simulink model "BatteryManagementSystem_V1"  (R2024a)
settings: Solver=VariableStepAuto  StartTime=0.0  StopTime=3600*2  RelTol=1e-3
InitFcn:
  | Capacity = 2.65;
  | c_rate= 0.5;
  | Np = 1; % Number of parallel cells
  | Ns = 3; % Number of series cells
  | voltageMin= 3.2;
  | currentThreshold = Capacity*Np/30;
  | voltageThreshold = 4.3;
  | CV_gain = 1;
  | voltageTolerance = 2;
undefined symbols (not defined in the file or in its folder): DiscIntNeverNeededParam
settings Model: Creator=MANSY  LastModifiedBy=MANSY
settings OptimizationCC: DefaultParameterBehavior=Inlined  UseDivisionForNetSlopeComputation=on  GainParamInheritBuiltInType=on  UseFloatMulNetSlope=on  InlineInvariantSignals=on  PassReuseOutputArgsAs=Individual arguments  ZeroExternalMemoryAtStartup=off  ZeroInternalMemoryAtStartup=off  NoFixptDivByZeroProtection=on  EfficientFloat2IntCast=on  LifeSpan=1  OptimizeBlockOrder=speed  DifferentSizesBufferReuse=on  EfficientTunableParamExpr=on
settings DebuggingCC: ParameterTunabilityLossMsg=error
settings HardwareCC: ProdBitPerInt=16  ProdBitPerPointer=16  ProdBitPerSizeT=16  ProdBitPerPtrDiffT=16  ProdLargestAtomicFloat=None  ProdWordSize=8  ProdLongLongMode=on  ProdHWDeviceType=Atmel->AVR
settings SFSimCC: MATLABDynamicMemAlloc=off
settings RTWCC: Description=Embedded Coder  SystemTargetFile=ert.tlc  TemplateMakefile=ert_default_tmf  PortableWordSizes=on
settings CodeAppCC: ForceParamTrailComments=on  IgnoreCustomStorageClasses=off  OperatorAnnotations=on  SimulinkDataObjDesc=on  SFDataObjDesc=on  CustomSymbolStrGlobalVar=rt$N$M  CustomSymbolStrType=$N$M  CustomSymbolStrFcn=$N$M$F  CustomSymbolStrMacro=$N$M  InsertBlockDesc=on
settings ERTTargetCC: TargetLangStandard=C99 (ISO)  GenerateSampleERTMain=on  IncludeMdlTerminateFcn=off  CombineSignalStateStructs=on  SupportComplex=off  SupportNonInlinedSFcns=on  InlinedParameterPlacement=NonHierarchical  ERTCustomFileTemplate=example_file_process.tlc  ERTFilePackagingFormat=CompactWithDataFile

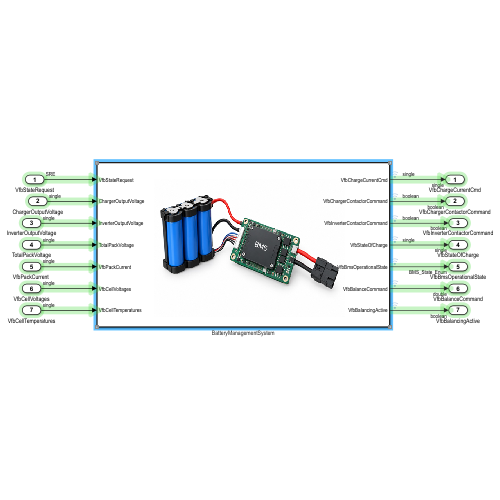
[thumbnail: Simulink's stored preview of the top-level diagram]
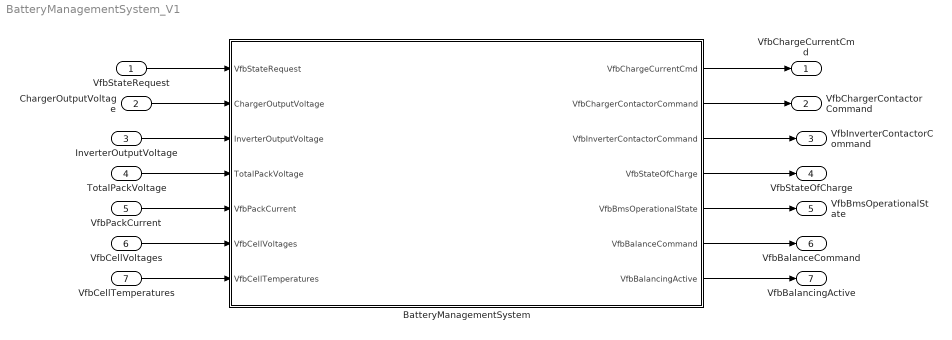
== system BatteryManagementSystem_V1 ==
  VfbStateRequest : Inport
  ChargerOutputVoltage : Inport  Port=2
  InverterOutputVoltage : Inport  Port=3
  TotalPackVoltage : Inport  Port=4
  "VfbPackCurrent " : Inport  Port=5
  VfbCellVoltages : Inport  Port=6
  VfbCellTemperatures : Inport  Port=7
  BatteryManagementSystem : Subsystem  TreatAsAtomicUnit=on
      mask Display: image('Lithium-Ion Battery BMS Module.png');
  VfbChargeCurrentCmd : Outport  OutDataTypeStr=single
  VfbChargerContactorCommand : Outport  Port=2  OutDataTypeStr=boolean
  VfbInverterContactorCommand : Outport  Port=3  OutDataTypeStr=boolean
  VfbStateOfCharge : Outport  Port=4  OutDataTypeStr=single
  VfbBmsOperationalState : Outport  Port=5
  VfbBalanceCommand : Outport  Port=6
  VfbBalancingActive : Outport  Port=7
  wires:
  VfbStateRequest/1 -> BatteryManagementSystem/1(VfbStateRequest)
  ChargerOutputVoltage/1 -> BatteryManagementSystem/2(ChargerOutputVoltage)
  InverterOutputVoltage/1 -> BatteryManagementSystem/3(InverterOutputVoltage)
  TotalPackVoltage/1 -> BatteryManagementSystem/4(TotalPackVoltage)
  "VfbPackCurrent "/1 -> BatteryManagementSystem/5("VfbPackCurrent ")
  VfbCellVoltages/1 -> BatteryManagementSystem/6(VfbCellVoltages)
  VfbCellTemperatures/1 -> BatteryManagementSystem/7(VfbCellTemperatures)
  BatteryManagementSystem/1(VfbChargeCurrentCmd) -> VfbChargeCurrentCmd/1
  BatteryManagementSystem/2(VfbChargerContactorCommand) -> VfbChargerContactorCommand/1
  BatteryManagementSystem/3(VfbInverterContactorCommand) -> VfbInverterContactorCommand/1
  BatteryManagementSystem/5(VfbBmsOperationalState) -> VfbBmsOperationalState/1
  BatteryManagementSystem/4(VfbStateOfCharge) -> VfbStateOfCharge/1
  BatteryManagementSystem/6(VfbBalanceCommand) -> VfbBalanceCommand/1
  BatteryManagementSystem/7(VfbBalancingActive) -> VfbBalancingActive/1

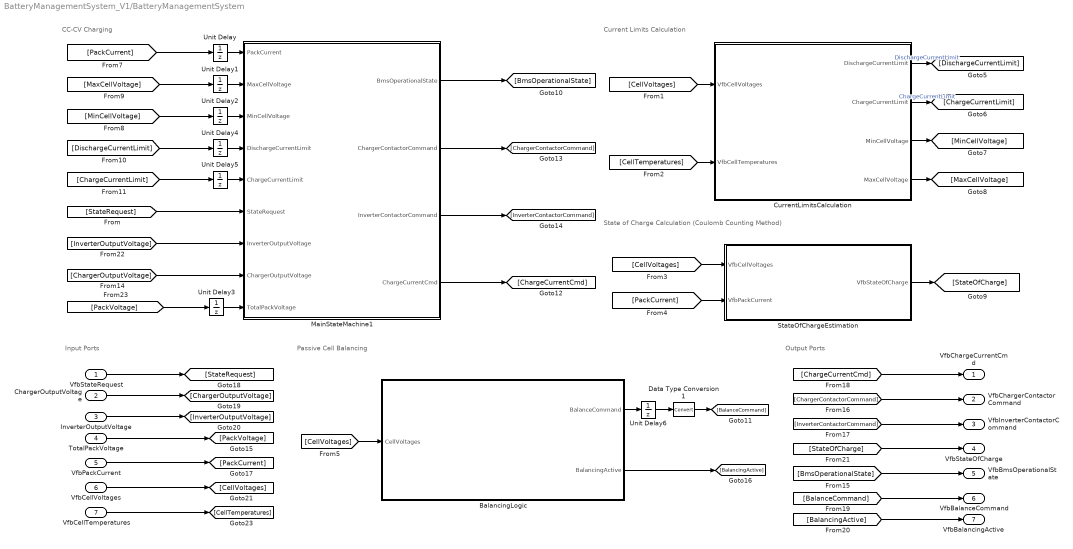
== system BatteryManagementSystem_V1/BatteryManagementSystem ==
  note: Passive Cell Balancing
  note: State of Charge Calculation (Coulomb Counting Method)
  note: Current Limits Calculation
  note: CC-CV Charging
  note: Output Ports
  note: Input Ports
  VfbStateRequest : Inport
  ChargerOutputVoltage : Inport  Port=2
  InverterOutputVoltage : Inport  Port=3
  TotalPackVoltage : Inport  Port=4
  "VfbPackCurrent " : Inport  Port=5
  VfbCellVoltages : Inport  Port=6
  VfbCellTemperatures : Inport  Port=7
  " StateOfChargeEstimation" : Subsystem  TreatAsAtomicUnit=on  SystemSampleTime=200e-3
      mask Display: image('SOC_img.png');
  BalancingLogic : MATLAB Function  TreatAsAtomicUnit=on  SystemSampleTime=250e-3
  "CurrentLimitsCalculation " : Subsystem  TreatAsAtomicUnit=on  SystemSampleTime=100e-3
      mask Display: image('CurrentLimit_img.png');
  Data Type Conversion1 : DataTypeConversion  SaturateOnIntegerOverflow=off  RndMeth=Floor
  MainStateMachine1 : Stateflow chart  TreatAsAtomicUnit=on  SystemSampleTime=50e-3
      settings: PortSchema="{\"entries\":[{\"content\":{\"sides\":[{\"content\":{\"connectorIds\":[\"In1\",\"In2\",\"In3\",\"In5\",\"In4\",\"In6\",\"In8\",\"In7\",\"In9\"]},\"type\":\"ConnectorPlacement.EquallySpacedRectSide\",\"uuid\":\"093f55e8-f90e-4d40-b8fb-904662301821\"},{\"content\":{\"connectorIds\":[\"Out1\",\"Out2\",\"Out3\",\"Out4\"],\"side\":\"RIGHT\"},\"type\":\"ConnectorPlacement.EquallySpacedRectSide\",\"uuid\":\"5101bd8f-b6b7-43f5-a647-8a1816a9003d\"},{\"content\":{\"side\":\"TOP\"},\"type\":\"ConnectorPlacement.EquallySpacedRectSide\",\"uuid\":\"c14aa96a-7f57-47da-866c-602a285b1131\"}]},\"type\":\"ConnectorPlacement.EquallySpacedConnector\",\"uuid\":\"8109f1a5-bcb4-40d5-94fc-489b7534b704\"}],\"packageUris\":[\"http://schema.mathworks.com/mf0/Connector/R2020b\"],\"version\":\"1.0\"}"
  Unit Delay{,1..6} (7 alike) : UnitDelay  SampleTime=-1  HasFrameUpgradeWarning=on
  VfbChargeCurrentCmd : Outport  OutDataTypeStr=single
  VfbChargerContactorCommand : Outport  Port=2  OutDataTypeStr=boolean
  VfbInverterContactorCommand : Outport  Port=3  OutDataTypeStr=boolean
  VfbStateOfCharge : Outport  Port=4  OutDataTypeStr=single
  VfbBmsOperationalState : Outport  Port=5
  VfbBalanceCommand : Outport  Port=6
  VfbBalancingActive : Outport  Port=7
  wires:
  TotalPackVoltage/1 -> [PackVoltage]
  MainStateMachine1/3(InverterContactorCommand) -> [InverterContactorCommand]
  [CellVoltages] -> "CurrentLimitsCalculation "/1(VfbCellVoltages)
  [BalancingActive] -> VfbBalancingActive/1
  "VfbPackCurrent "/1 -> [PackCurrent]
  "CurrentLimitsCalculation "/4(MaxCellVoltage) -> [MaxCellVoltage]
  [StateOfCharge] -> VfbStateOfCharge/1
  [InverterContactorCommand] -> VfbInverterContactorCommand/1
  [PackCurrent] -> Unit Delay/1
  MainStateMachine1/4(ChargeCurrentCmd) -> [ChargeCurrentCmd]
  Unit Delay5/1 -> MainStateMachine1/4(ChargeCurrentLimit)
  Data Type Conversion1/1 -> [BalanceCommand]
  [BalanceCommand] -> VfbBalanceCommand/1
  [ChargerContactorCommand] -> VfbChargerContactorCommand/1
  [InverterOutputVoltage] -> MainStateMachine1/8(InverterOutputVoltage)
  Unit Delay3/1 -> MainStateMachine1/9(TotalPackVoltage)
  [BmsOperationalState] -> VfbBmsOperationalState/1
  [StateRequest] -> MainStateMachine1/6(StateRequest)
  BalancingLogic/1(BalanceCommand) -> Unit Delay6/1
  BalancingLogic/2(BalancingActive) -> [BalancingActive]
  [DischargeCurrentLimit] -> Unit Delay4/1
  [ChargeCurrentCmd] -> VfbChargeCurrentCmd/1
  [ChargerOutputVoltage] -> MainStateMachine1/7(ChargerOutputVoltage)
  [ChargeCurrentLimit] -> Unit Delay5/1
  Unit Delay/1 -> MainStateMachine1/1(PackCurrent)
  Unit Delay1/1 -> MainStateMachine1/2(MaxCellVoltage)
  [CellTemperatures] -> "CurrentLimitsCalculation "/2(VfbCellTemperatures)
  [PackCurrent] -> " StateOfChargeEstimation"/2("VfbPackCurrent ")
  InverterOutputVoltage/1 -> [InverterOutputVoltage]
  Unit Delay6/1 -> Data Type Conversion1/1
  MainStateMachine1/2(ChargerContactorCommand) -> [ChargerContactorCommand]
  [MaxCellVoltage] -> Unit Delay1/1
  VfbCellVoltages/1 -> [CellVoltages]
  [PackVoltage] -> Unit Delay3/1
  VfbCellTemperatures/1 -> [CellTemperatures]
  [CellVoltages] -> BalancingLogic/1(CellVoltages)
  [CellVoltages] -> " StateOfChargeEstimation"/1(VfbCellVoltages)
  MainStateMachine1/1(BmsOperationalState) -> [BmsOperationalState]
  [MinCellVoltage] -> Unit Delay2/1
  "CurrentLimitsCalculation "/2(ChargeCurrentLimit) -> [ChargeCurrentLimit]  "ChargeCurrentLimit"
  ChargerOutputVoltage/1 -> [ChargerOutputVoltage]
  "CurrentLimitsCalculation "/1(DischargeCurrentLimit) -> [DischargeCurrentLimit]  "DischargeCurrentLimit"
  " StateOfChargeEstimation"/1(VfbStateOfCharge) -> [StateOfCharge]
  Unit Delay4/1 -> MainStateMachine1/5(DischargeCurrentLimit)
  VfbStateRequest/1 -> [StateRequest]
  Unit Delay2/1 -> MainStateMachine1/3(MinCellVoltage)
  "CurrentLimitsCalculation "/3(MinCellVoltage) -> [MinCellVoltage]

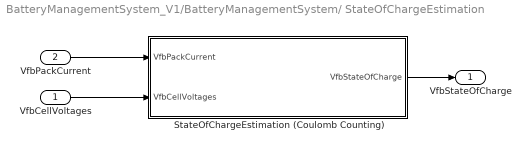
== system BatteryManagementSystem_V1/BatteryManagementSystem/ StateOfChargeEstimation ==
  VfbCellVoltages : Inport
  "VfbPackCurrent " : Inport  Port=2
  StateOfChargeEstimation (Coulomb Counting) : Subsystem  TreatAsAtomicUnit=on
  VfbStateOfCharge : Outport
  wires:
  StateOfChargeEstimation (Coulomb Counting)/1(VfbStateOfCharge) -> VfbStateOfCharge/1
  "VfbPackCurrent "/1 -> StateOfChargeEstimation (Coulomb Counting)/1("VfbPackCurrent ")
  VfbCellVoltages/1 -> StateOfChargeEstimation (Coulomb Counting)/2(VfbCellVoltages)

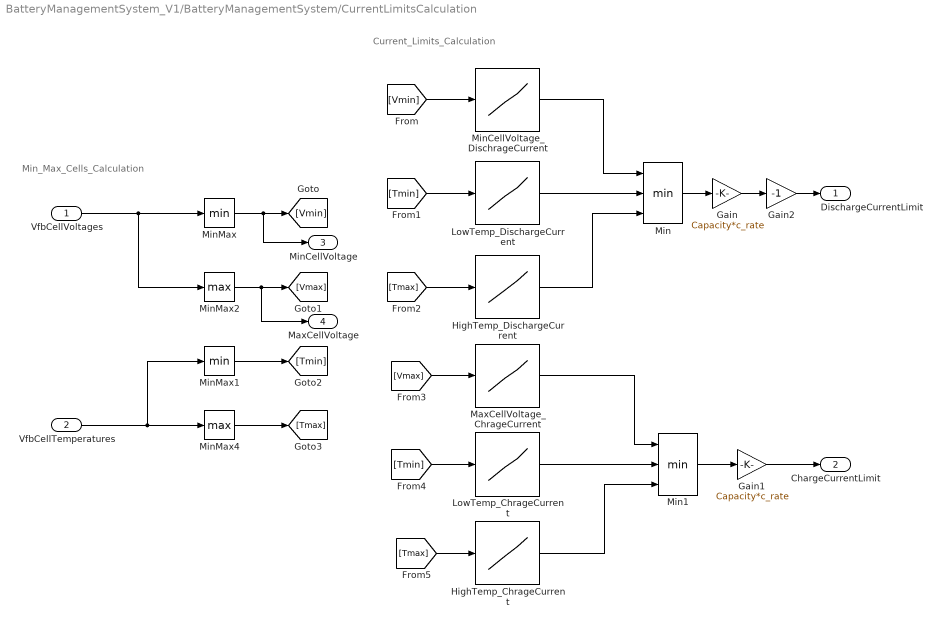
== system BatteryManagementSystem_V1/BatteryManagementSystem/CurrentLimitsCalculation  ==
  note: Current_Limits_Calculation
  note: Min_Max_Cells_Calculation
  VfbCellVoltages : Inport  OutDataTypeStr=single  PortDimensions=3
  VfbCellTemperatures : Inport  Port=2  OutDataTypeStr=single  PortDimensions=3
  Gain : Gain  Gain=Capacity*c_rate
  Gain1 : Gain  Gain=Capacity*c_rate
  Gain2 : Gain  Gain=-1
  HighTemp_ChrageCurrent : Lookup_n-D  NumberOfTableDimensions=1  BreakpointsForDimension1=single([298.15 308.15 313.15 318.15 323.15 333.15])  Table=single([1 1 0.8 0.5 0.2 0])  InternalRulePriority=Speed  RndMeth=Simplest
  HighTemp_DischargeCurrent : Lookup_n-D  NumberOfTableDimensions=1  BreakpointsForDimension1=single([298.15 308.15 313.15 318.15 323.15 333.15])  Table=single([1 1 0.9 0.7 0.4 0])  InternalRulePriority=Speed  RndMeth=Simplest
  LowTemp_ChrageCurrent : Lookup_n-D  NumberOfTableDimensions=1  BreakpointsForDimension1=single([243.15 263.15 273.15 278.15 283.15 288.15 298.15])  Table=single([0 0 0 0.1 0.3 0.6 1])  InternalRulePriority=Speed  RndMeth=Simplest
  LowTemp_DischargeCurrent : Lookup_n-D  NumberOfTableDimensions=1  BreakpointsForDimension1=single([243.15 258.15 273.15 283.15 293.15 298.15])  Table=single([0 0 0.2 0.6 0.9 1])  InternalRulePriority=Speed  RndMeth=Simplest
  MaxCellVoltage_ChrageCurrent : Lookup_n-D  NumberOfTableDimensions=1  BreakpointsForDimension1=single([3.0 3.5 3.8 4.0 4.1 4.2 4.25 4.35])  Table=single([1 1 1 0.9 0.7 0.4 0.2 0])  InternalRulePriority=Speed  RndMeth=Simplest
  Min : MinMax  Inputs=3
  Min1 : MinMax  Inputs=3
  MinCellVoltage_DischrageCurrent : Lookup_n-D  NumberOfTableDimensions=1  BreakpointsForDimension1=single([2.7 2.8 3.0 3.2 3.4 3.6])  Table=single([0 0.1 0.3 0.6 0.9 1])  InternalRulePriority=Speed  RndMeth=Simplest
  MinMax : MinMax
  MinMax1 : MinMax
  MinMax2 : MinMax  Function=max
  MinMax4 : MinMax  Function=max
  DischargeCurrentLimit : Outport  OutDataTypeStr=single
  ChargeCurrentLimit : Outport  Port=2  OutDataTypeStr=single
  MinCellVoltage : Outport  Port=3
  MaxCellVoltage : Outport  Port=4
  wires:
  [Vmin] -> MinCellVoltage_DischrageCurrent/1
  Gain/1 -> Gain2/1
  VfbCellVoltages/1 -> MinMax2/1, MinMax/1
  LowTemp_ChrageCurrent/1 -> Min1/2
  [Tmin] -> LowTemp_ChrageCurrent/1
  MinMax4/1 -> [Tmax]
  [Tmin] -> LowTemp_DischargeCurrent/1
  [Tmax] -> HighTemp_ChrageCurrent/1
  Min1/1 -> Gain1/1
  MaxCellVoltage_ChrageCurrent/1 -> Min1/1
  MinMax/1 -> MinCellVoltage/1, [Vmin]
  LowTemp_DischargeCurrent/1 -> Min/2
  MinMax2/1 -> MaxCellVoltage/1, [Vmax]
  HighTemp_DischargeCurrent/1 -> Min/3
  HighTemp_ChrageCurrent/1 -> Min1/3
  Gain1/1 -> ChargeCurrentLimit/1
  [Tmax] -> HighTemp_DischargeCurrent/1
  Min/1 -> Gain/1
  [Vmax] -> MaxCellVoltage_ChrageCurrent/1
  MinCellVoltage_DischrageCurrent/1 -> Min/1
  VfbCellTemperatures/1 -> MinMax4/1, MinMax1/1
  MinMax1/1 -> [Tmin]
  Gain2/1 -> DischargeCurrentLimit/1

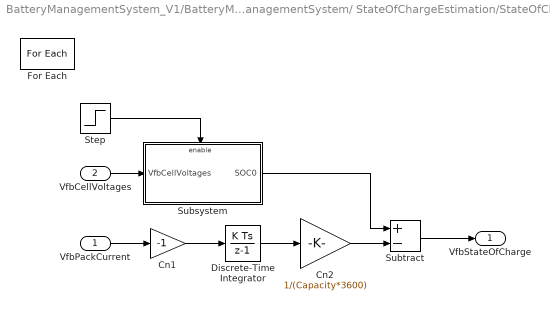
== system BatteryManagementSystem_V1/BatteryManagementSystem/ StateOfChargeEstimation/StateOfChargeEstimation (Coulomb Counting) ==
  "VfbPackCurrent " : Inport  OutDataTypeStr=single
  VfbCellVoltages : Inport  Port=2  Partition=on  PartitionDimension=1  PartitionWidth=1  PartitionOffset=0
  Cn1 : Gain  Gain=-1  OutDataTypeStr=single
  Cn2 : Gain  Gain=1/(Capacity*3600)  OutDataTypeStr=single
  Discrete-Time Integrator : DiscreteIntegrator  gainval=1  SampleTime=-1  OutDataTypeStr=single  RndMeth=Nearest  ICPrevOutput=DiscIntNeverNeededParam  ICPrevScaledInput=DiscIntNeverNeededParam
  For Each : ForEach  DisableCoverage=on
  Step : Step  Time=0.1  Before=1  After=0
  Subsystem : Subsystem
  Subtract : Sum  Inputs=+-
  VfbStateOfCharge : Outport  OutDataTypeStr=single  ConcatenationDimension=1
  wires:
  Cn1/1 -> Discrete-Time Integrator/1
  Discrete-Time Integrator/1 -> Cn2/1
  "VfbPackCurrent "/1 -> Cn1/1
  Subtract/1 -> VfbStateOfCharge/1
  Subsystem/1(SOC0) -> Subtract/1
  Step/1 -> Subsystem/Enable
  VfbCellVoltages/1 -> Subsystem/1(VfbCellVoltages)
  Cn2/1 -> Subtract/2

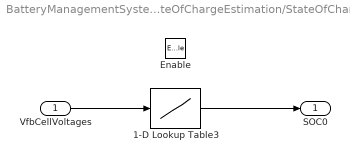
== system BatteryManagementSystem_V1/BatteryManagementSystem/ StateOfChargeEstimation/StateOfChargeEstimation (Coulomb Counting)/Subsystem ==
  VfbCellVoltages : Inport
  Enable : EnablePort
  1-D Lookup Table3 : Lookup_n-D  NumberOfTableDimensions=1  BreakpointsForDimension1=|  Table=|  InternalRulePriority=Speed  RndMeth=Simplest
      BreakpointsForDimension1=|
      | [3.04339, 3.19969, 3.32733, 3.41897, 3.47789, 3.5189, ...
      | 3.54757, 3.56926, 3.58543, 3.59715, 3.60656, 3.61458, ...
      | 3.62125, 3.62859, 3.63585, 3.64117, 3.64677, 3.65281, ...
      | 3.65754, 3.6622, 3.66686, 3.67118, 3.67547, 3.67953, ...
      | 3.68333, 3.68679, 3.68929, 3.69163, 3.69398, 3.69633, ...
      | 3.69868, 3.70108, 3.7035, 3.70592, 3.70834, 3.71076, ...
      | 3.71334, 3.71599, 3.71889, 3.72198, 3.72508, 3.72817, ...
      | 3.73126, 3.73436, 3.73745, 3.74054, 3.74364, 3.74686, ...
      | 3.75011, 3.75346, 3.75768, 3.7621, 3.76652, 3.77094, ...
      | 3.77575, 3.78058, 3.78546, 3.79147, 3.79777, 3.80409, ...
      | 3.8104, 3.81672, 3.82303, 3.82935, 3.83618, 3.84344, ...
      | 3.8508, 3.85816, 3.86553, 3.87289, 3.88052, 3.88833, ...
      | 3.89603, 3.90423, 3.91256, 3.92124, 3.93029, 3.93933, ...
      | 3.94837, 3.95788, 3.96788, 3.97854, 3.98931, 4.00008, ...
      | 4.01149, 4.02304, 4.03459, 4.04614, 4.05768, 4.06947, ...
      | 4.08184, 4.09422, 4.1067, 4.11982, 4.1326, 4.14615, ...
      | 4.15754, 4.16699, 4.17222, 4.18119, 4.30838]
      Table=|
      | [0, 0.01, 0.02, 0.03, 0.04, 0.05, 0.06, 0.07, 0.08, 0.09, ...
      | 0.10, 0.11, 0.12, 0.13, 0.14, 0.15, 0.16, 0.17, 0.18, 0.19, ...
      | 0.20, 0.21, 0.22, 0.23, 0.24, 0.25, 0.26, 0.27, 0.28, 0.29, ...
      | 0.30, 0.31, 0.32, 0.33, 0.34, 0.35, 0.36, 0.37, 0.38, 0.39, ...
      | 0.40, 0.41, 0.42, 0.43, 0.44, 0.45, 0.46, 0.47, 0.48, 0.49, ...
      | 0.50, 0.51, 0.52, 0.53, 0.54, 0.55, 0.56, 0.57, 0.58, 0.59, ...
      | 0.60, 0.61, 0.62, 0.63, 0.64, 0.65, 0.66, 0.67, 0.68, 0.69, ...
      | 0.70, 0.71, 0.72, 0.73, 0.74, 0.75, 0.76, 0.77, 0.78, 0.79, ...
      | 0.80, 0.81, 0.82, 0.83, 0.84, 0.85, 0.86, 0.87, 0.88, 0.89, ...
      | 0.90, 0.91, 0.92, 0.93, 0.94, 0.95, 0.96, 0.97, 0.98, 0.99, 1]
  SOC0 : Outport
  wires:
  VfbCellVoltages/1 -> 1-D Lookup Table3/1
  1-D Lookup Table3/1 -> SOC0/1

== stateflow chart BatteryManagementSystem_V1/BatteryManagementSystem/MainStateMachine1 ==
  state Charging
    entry:
    BmsOperationalState = BMS_State_Enum.Charging;
    ChargerContactorCommand =1;
    exit:
    ChargerContactorCommand =0;
    state CC
      entry:
      ChargeCurrentCmd = ChargeCurrentLimit;
    state CV
      during:
      ChargeCurrentCmd = ChargeCurrentCmd - CV_gain*(MaxCellVoltage - voltageThreshold);
      ChargeCurrentCmd = min(ChargeCurrentCmd, ChargeCurrentLimit);
    (default) -> CC
    CC -> CV : [MaxCellVoltage > voltageThreshold]
  state Discharging
    entry:
    InverterContactorCommand = 1;
    BmsOperationalState = BMS_State_Enum.Discharging;
    during:
    ChargeCurrentCmd = DischargeCurrentLimit;
    exit:
    InverterContactorCommand = 0;
  state Standby
    entry:
    ChargeCurrentCmd = 0;
    BmsOperationalState = BMS_State_Enum.Standby;
    InverterContactorCommand =0;
    ChargerContactorCommand =0;
  Discharging -> Charging [order 1] : [StateRequest ==	SRE.SRE_Charging && abs(ChargerOutputVoltage - TotalPackVoltage) < voltageTolerance]
  Charging -> Discharging [order 2] : [StateRequest ==	SRE.SRE_Discharging && abs(InverterOutputVoltage - TotalPackVoltage ) < voltageTolerance && abs(ChargerOutputVoltage - TotalPackVoltage) < voltageTolerance]
  Standby -> Discharging [order 1] : [(StateRequest ==	SRE.SRE_Discharging) && (MinCellVoltage > 1.1*voltageMin) && (abs(InverterOutputVoltage - TotalPackVoltage ) < voltageTolerance) ]
  Discharging -> Standby [order 2] : [ StateRequest ==	SRE.SRE_Standby || MinCellVoltage < voltageMin ]
  (default) -> Standby
  Charging -> Standby [order 1] : [ StateRequest ==	SRE.SRE_Standby || PackCurrent < currentThreshold ]
  Standby -> Charging [order 2] : [StateRequest ==	SRE.SRE_Charging && MinCellVoltage < 0.95*voltageThreshold && abs(ChargerOutputVoltage - TotalPackVoltage) < voltageTolerance]
  data: CV_gain parameter single; currentThreshold parameter single; voltageMin parameter single; voltageThreshold parameter single; PackCurrent input single; MaxCellVoltage input single; MinCellVoltage input single; ChargeCurrentLimit input single; DischargeCurrentLimit input single; StateRequest input Enum: SRE; BmsOperationalState output Enum: BMS_State_Enum; voltageTolerance parameter single; ChargerOutputVoltage input single; InverterOutputVoltage input single; TotalPackVoltage input single; ChargerContactorCommand output boolean; InverterContactorCommand output boolean; ChargeCurrentCmd output single

== matlab function BatteryManagementSystem_V1/BatteryManagementSystem/BalancingLogic ==
  data: CellVoltages input; BalanceCommand output boolean; BalancingActive output
function [BalanceCommand,BalancingActive]= fcn(CellVoltages)
Vmin = min(CellVoltages);
BalanceCommand = false(size(CellVoltages));
BalancingActive = false;
deltaV_threshold = 0.05;
for i = 1: length(CellVoltages)
   deltaV = CellVoltages(i)-Vmin;
   BalanceCommand(i) = deltaV >deltaV_threshold;
end

BalancingActive = any(BalanceCommand);

end
